simulink model "LQR_simulation"  (R2025a)
settings: Solver=ode4  StartTime=0.0  StopTime=200  FixedStep=0.001  RelTol=1e-3
values from neighbouring files (symbols this model uses):
  K = lqr(A, B, Q, R)    [LQR_design.m]
  x_target = [0; 1; 0]    [LQR_design.m]
undefined symbols (not defined in the file or in its folder): p
settings Model: Creator=Giammo  LastModifiedBy=Giammo

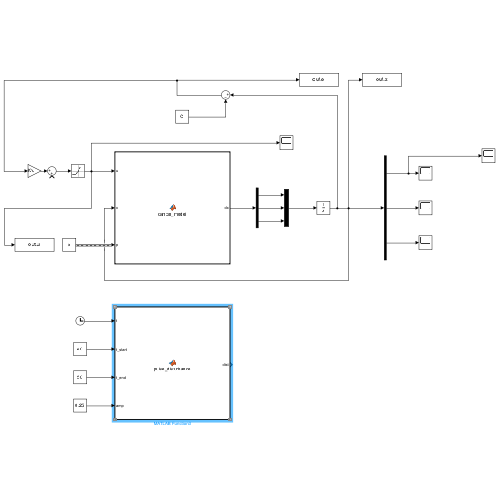
[thumbnail: Simulink's stored preview of the top-level diagram]
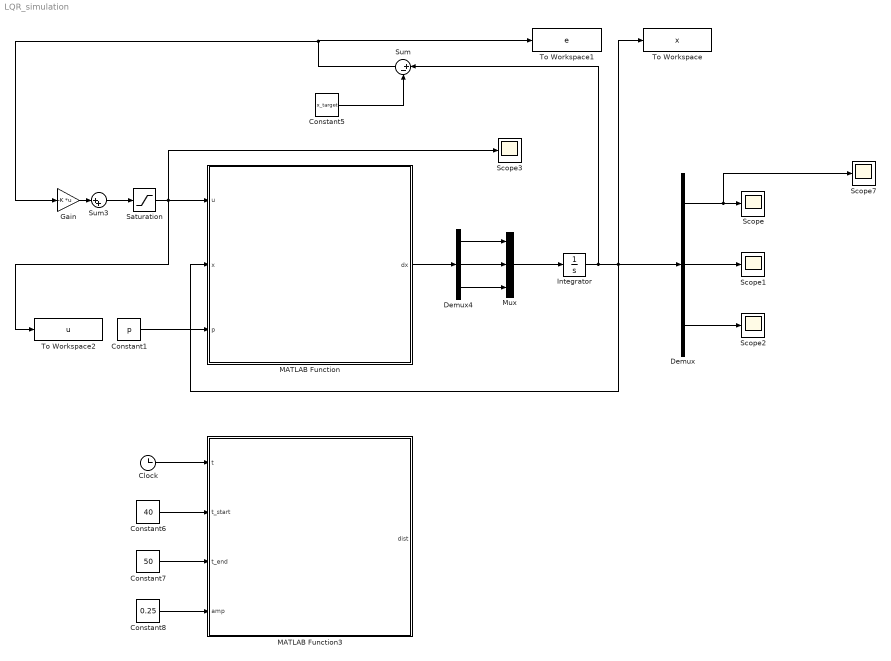
== system LQR_simulation ==
  Clock : Clock
  Constant1 : Constant  Value=p  OutDataTypeStr=Bus: slBus1
  Constant5 : Constant  Value=x_target
  Constant6 : Constant  Value=40
  Constant7 : Constant  Value=50
  Constant8 : Constant  Value=0.25
  Demux : Demux  Outputs=3
  Demux4 : Demux  Outputs=3
  Gain : Gain  Gain=-K  Multiplication=Matrix(K*u)
  Integrator : Integrator  InitialCondition=[0.1;0.1;0.1]  UpperSaturationLimit=1  LowerSaturationLimit=[0;0;0]
  MATLAB Function : MATLAB Function  TreatAsAtomicUnit=on
  MATLAB Function3 : MATLAB Function  TreatAsAtomicUnit=on
  Mux : Mux  Inputs=3
  Saturation : Saturate  UpperLimit=1  LowerLimit=0
  Scope{,1..3,7} (5 alike) : Scope
      Scope settings: ActiveDisplayYMinimum=0.0015797842049656216  ActiveDisplayYMaximum=0.12471331968367572
      Scope1 settings: ActiveDisplayYMinimum=-0.0012214326520152419  ActiveDisplayYMaximum=1.0109928938681374
      Scope2 settings: ActiveDisplayYMinimum=-0.12960308023687167  ActiveDisplayYMaximum=1.1908049530763261  DataLoggingVariableName=ScopeData2
      Scope3 settings: ActiveDisplayYMinimum=-0.017719033674089384  ActiveDisplayYMaximum=0.17228053017196643  DataLoggingVariableName=ScopeData3
      Scope7 settings: ActiveDisplayYMinimum=-0.10710642652310215  ActiveDisplayYMaximum=1.0119007140581224  DataLoggingVariableName=ScopeData7
  Sum : Sum  Inputs=|+-
  Sum3 : Sum  Inputs=|++
  To Workspace : ToWorkspace  VariableName=x  SaveFormat=Timeseries  SampleTime=-1
  To Workspace1 : ToWorkspace  VariableName=e  SaveFormat=Timeseries  SampleTime=-1
  To Workspace2 : ToWorkspace  VariableName=u  SaveFormat=Timeseries  SampleTime=-1
  wires:
  Integrator/1 -> Sum/1, To Workspace/1, Demux/1, MATLAB Function/2(x)
  Demux/1 -> Scope7/1, Scope/1
  Demux/2 -> Scope1/1
  Demux/3 -> Scope2/1
  Constant1/1 -> MATLAB Function/3(p)
  Constant5/1 -> Sum/2
  Sum/1 -> To Workspace1/1, Gain/1
  Sum3/1 -> Saturation/1
  MATLAB Function/1(dx) -> Demux4/1
  Demux4/2 -> Mux/2
  Mux/1 -> Integrator/1
  Clock/1 -> MATLAB Function3/1(t)
  Constant7/1 -> MATLAB Function3/3(t_end)
  Constant6/1 -> MATLAB Function3/2(t_start)
  Constant8/1 -> MATLAB Function3/4(amp)
  Gain/1 -> Sum3/1
  Demux4/1 -> Mux/1
  Demux4/3 -> Mux/3
  Saturation/1 -> MATLAB Function/1(u), Scope3/1, To Workspace2/1

== matlab function LQR_simulation/MATLAB Function ==
  data: u input; dx output; x input; p input
function dx = cancer_model(u, x, p)
    % Continuous-time dynamics: states are tumor, hunting cells and resting cells; u acts on x3.

    x1 = x(1);
    x2 = x(2);
    x3 = x(3);
    A12 = p.A12;
    A13 = p.A13;
    R2  = p.R2;
    A21 = p.A21;
    R3  = p.R3;
    k3  = p.k3;
    A31 = p.A31;
    D3  = p.D3;
    dx = zeros(3,1);
    dx(1) = x1*(1 - x1) - A12*x1*x2 - A13*x1*x3;
    dx(2) = R2*x2*(1 - x2) - A21*x1*x2;
    recruitment = (R3 * x1 * x3) / (x1 + k3);
    dx(3) = recruitment - A31*x1*x3 - D3*x3 + u;

end

== matlab function LQR_simulation/MATLAB Function3 ==
  data: t input; dist output; t_start input; t_end input; amp input
function dist = pulse_disturbance(t, t_start, t_end, amp)
    % Apply a constant disturbance during the selected time interval.


    if (t >= t_start && t <= t_end)
        dist = amp;
    else
        dist = 0;
    end
    
end
